simulink subsystem "cmac2d"  (R2024b)
settings: Solver=VariableStepAuto  StartTime=0.0  StopTime=10.0  RelTol=1e-3
undefined symbols (not defined in the file): Cin, Cout, L, LOG2L, NKEEP
libraries: hdlsllib x12
settings Model: Creator=User  LastModifiedBy=User

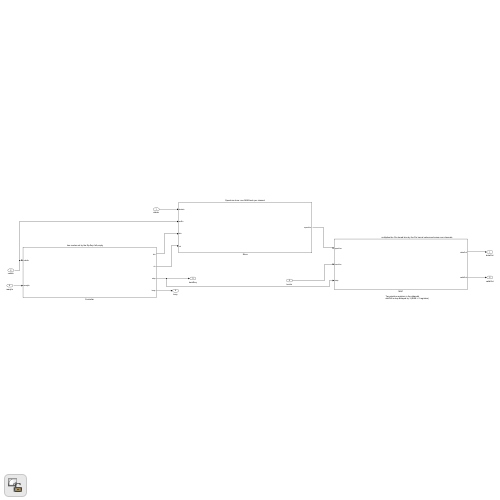
[thumbnail: Simulink's stored preview of the top-level diagram]
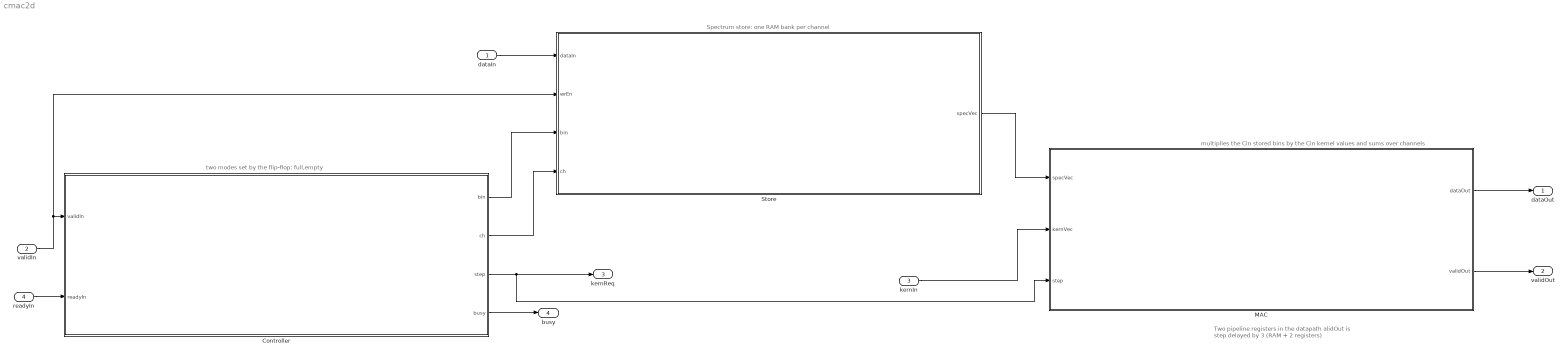
== system cmac2d ==
  note: two modes set by the flip-flop: full,empty
  note: Spectrum store: one RAM bank per channel
  note: multiplies the Cin stored bins by the Cin kernel values and sums over channels
  note: Two pipeline registers in the datapath
      | alidOut is step delayed by 3 (RAM + 2 registers)
  dataIn : Inport  OutDataTypeStr=fixdt(1,23,0)
      settings: SignalType=complex
  validIn : Inport  Port=2
  kernIn : Inport  Port=3  OutDataTypeStr=fixdt(1,KERN_WL,0)  PortDimensions=Cin
      settings: SignalType=complex
  readyIn : Inport  Port=4
  Controller : Subsystem
  MAC : Subsystem
  Store : Subsystem
  dataOut : Outport
  validOut : Outport  Port=2
  kernReq : Outport  Port=3
  busy : Outport  Port=4
  wires:
  Controller/3(step) -> kernReq/1, MAC/3(step)
  kernIn/1 -> MAC/2(kernVec)
  readyIn/1 -> Controller/2(readyIn)
  dataIn/1 -> Store/1(dataIn)
  validIn/1 -> Controller/1(validIn), Store/2(wrEn)
  Controller/1(bin) -> Store/3(bin)
  Controller/2(ch) -> Store/4(ch)
  Controller/4(busy) -> busy/1
  Store/1(specVec) -> MAC/1(specVec)
  MAC/1(dataOut) -> dataOut/1
  MAC/2(validOut) -> validOut/1

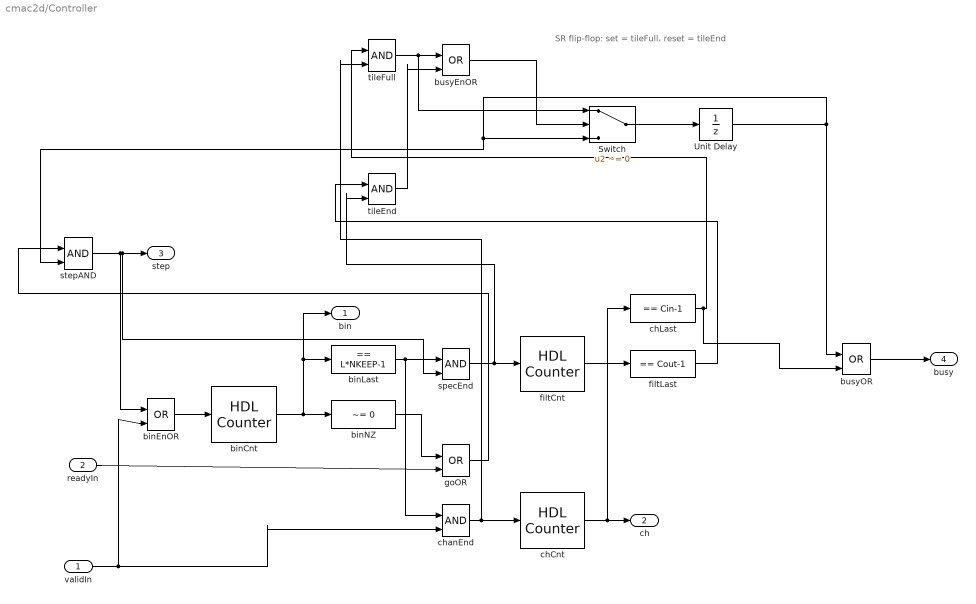
== system cmac2d/Controller ==
  note: SR flip-flop: set = tileFull، reset = tileEnd
  validIn : Inport
  readyIn : Inport  Port=2
  Switch : Switch  Criteria=u2 ~= 0  SaturateOnIntegerOverflow=off  InputSameDT=off
  Unit Delay : UnitDelay  SampleTime=-1  HasFrameUpgradeWarning=on
  binCnt : hdlsllib/Sources/HDL Counter  CountType=Count limited  CountInit=0  CountStep=1  CountMax=L*NKEEP-1  CountFromType=Initial value  CountFrom=0  CountResetPort=off  CountLoadPort=off  CountEnbPort=on  CountDirPort=off  CountHitOutputPort=off  CountDataType=Unsigned  CountWordLen=2*LOG2L  CountFracLen=0  CountSampTime=1
  binEnOR : Logic  Operator=OR  IconShape=distinctive  AllPortsSameDT=off  OutDataTypeStr=boolean
  binLast : hdlsllib/Logic and Bit Operations/Compare To Constant  relop===  const=L*NKEEP-1  OutDataTypeStr=boolean
  binNZ : hdlsllib/Logic and Bit Operations/Compare To Constant  relop=~=  const=0  OutDataTypeStr=boolean
  busyEnOR : Logic  Operator=OR  IconShape=distinctive  AllPortsSameDT=off  OutDataTypeStr=boolean
  busyOR : Logic  Operator=OR  IconShape=distinctive  AllPortsSameDT=off  OutDataTypeStr=boolean
  chCnt : hdlsllib/Sources/HDL Counter  CountType=Count limited  CountInit=0  CountStep=1  CountMax=Cin-1  CountFromType=Initial value  CountFrom=0  CountResetPort=off  CountLoadPort=off  CountEnbPort=on  CountDirPort=off  CountHitOutputPort=off  CountDataType=Unsigned  CountWordLen=ceil(log2(Cin))  CountFracLen=0  CountSampTime=1
  chLast : hdlsllib/Logic and Bit Operations/Compare To Constant  relop===  const=Cin-1  OutDataTypeStr=boolean
  chanEnd : Logic  IconShape=distinctive  AllPortsSameDT=off  OutDataTypeStr=boolean
  filtCnt : hdlsllib/Sources/HDL Counter  CountType=Count limited  CountInit=0  CountStep=1  CountMax=Cout-1  CountFromType=Initial value  CountFrom=0  CountResetPort=off  CountLoadPort=off  CountEnbPort=on  CountDirPort=off  CountHitOutputPort=off  CountDataType=Unsigned  CountWordLen=ceil(log2(Cout))  CountFracLen=0  CountSampTime=1
  filtLast : hdlsllib/Logic and Bit Operations/Compare To Constant  relop===  const=Cout-1  OutDataTypeStr=boolean
  goOR : Logic  Operator=OR  IconShape=distinctive  AllPortsSameDT=off  OutDataTypeStr=boolean
  specEnd : Logic  IconShape=distinctive  AllPortsSameDT=off  OutDataTypeStr=boolean
  stepAND : Logic  IconShape=distinctive  AllPortsSameDT=off  OutDataTypeStr=boolean
  tileEnd : Logic  IconShape=distinctive  AllPortsSameDT=off  OutDataTypeStr=boolean
  tileFull : Logic  IconShape=distinctive  AllPortsSameDT=off  OutDataTypeStr=boolean
  bin : Outport
  ch : Outport  Port=2
  step : Outport  Port=3
  busy : Outport  Port=4
  wires:
  busyOR/1 -> busy/1
  filtLast/1 -> tileEnd/1
  chLast/1 -> tileFull/1, busyOR/2
  chCnt/1 -> chLast/1, ch/1
  Switch/1 -> Unit Delay/1
  chanEnd/1 -> chCnt/1, tileFull/2
  busyEnOR/1 -> Switch/2
  goOR/1 -> stepAND/1
  readyIn/1 -> goOR/2
  binNZ/1 -> goOR/1
  tileEnd/1 -> busyEnOR/2
  tileFull/1 -> busyEnOR/1, Switch/1
  Unit Delay/1 -> stepAND/2, Switch/3, busyOR/1
  validIn/1 -> binEnOR/2, chanEnd/2
  specEnd/1 -> filtCnt/1, tileEnd/2
  binCnt/1 -> binNZ/1, bin/1, binLast/1
  binEnOR/1 -> binCnt/1
  binLast/1 -> chanEnd/1, specEnd/1
  stepAND/1 -> binEnOR/1, step/1, specEnd/2
  filtCnt/1 -> filtLast/1

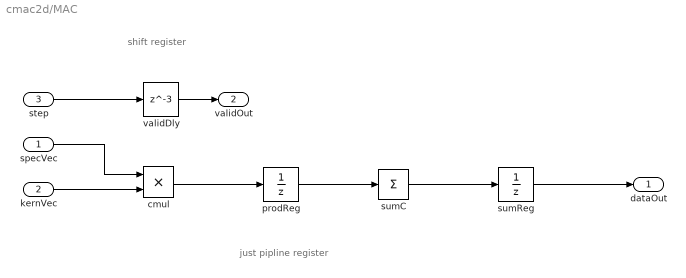
== system cmac2d/MAC ==
  note: just pipline register
  note: shift register
  specVec : Inport
  kernVec : Inport  Port=2
  step : Inport  Port=3
  cmul : Product  OutDataTypeStr=fixdt(1,X_WL+KERN_WL+1,0)
  prodReg : UnitDelay  SampleTime=-1  HasFrameUpgradeWarning=on
  sumC : Sum  Inputs=+  OutDataTypeStr=fixdt(1,X_WL+KERN_WL+1+ceil(log2(Cin)),0)
  sumReg : UnitDelay  SampleTime=-1  HasFrameUpgradeWarning=on
  validDly : Delay  DelayLength=3  InitialCondition=0
  dataOut : Outport
  validOut : Outport  Port=2
  wires:
  sumReg/1 -> dataOut/1
  prodReg/1 -> sumC/1
  validDly/1 -> validOut/1
  cmul/1 -> prodReg/1
  kernVec/1 -> cmul/2
  sumC/1 -> sumReg/1
  specVec/1 -> cmul/1
  step/1 -> validDly/1

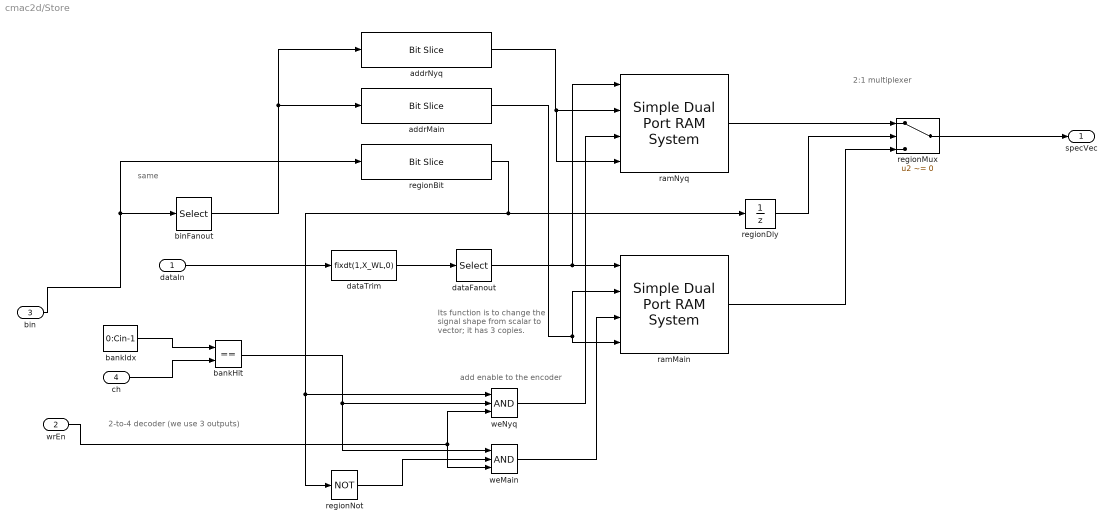
== system cmac2d/Store ==
  note: 2-to-4 decoder (we use 3 outputs)
  note: add enable to the encoder
  note: 2:1 multiplexer
  note: Its function is to change
      | the signal shape
      | from scalar to vector;
      |  it has 3 copies.
  note: same
  dataIn : Inport  PortDimensions=1
  wrEn : Inport  Port=2
  bin : Inport  Port=3
  ch : Inport  Port=4
  addrMain : hdlsllib/Logic and Bit Operations/Bit Slice  lidx=2*LOG2L-2  ridx=0
  addrNyq : hdlsllib/Logic and Bit Operations/Bit Slice  lidx=LOG2L-1  ridx=0
  bankHit : RelationalOperator  Operator===  OutDataTypeStr=boolean  InputSameDT=off
  bankIdx : Constant  Value=0:Cin-1  OutDataTypeStr=fixdt(0,ceil(log2(Cin)),0)
  binFanout : Selector  InputPortWidth=1  IndexOptions=Index vector (dialog)  Indices=ones(1,Cin)  OutputSizes=1
  dataFanout : Selector  InputPortWidth=1  IndexOptions=Index vector (dialog)  Indices=ones(1,Cin)  OutputSizes=1
  dataTrim : DataTypeConversion  OutDataTypeStr=fixdt(1,X_WL,0)  SaturateOnIntegerOverflow=off  RndMeth=Floor
  ramMain : hdlsllib/HDL RAMs/Simple Dual Port RAM System  RAMType=Simple dual port  AsyncRead=off  WriteOutputValue=New data  RAMInitialValue=0  allowBusInputs=off  WritesHaveOutput=on  NumReads=0  NumWrites=1  SimulateUsing=Code generation  ModelRAMDelay=on
  ramNyq : hdlsllib/HDL RAMs/Simple Dual Port RAM System  RAMType=Simple dual port  AsyncRead=off  WriteOutputValue=New data  RAMInitialValue=0  allowBusInputs=off  WritesHaveOutput=on  NumReads=0  NumWrites=1  SimulateUsing=Code generation  ModelRAMDelay=on
  regionBit : hdlsllib/Logic and Bit Operations/Bit Slice  lidx=2*LOG2L-1  ridx=2*LOG2L-1
  regionDly : UnitDelay  SampleTime=-1  HasFrameUpgradeWarning=on
  regionMux : Switch  Criteria=u2 ~= 0  SaturateOnIntegerOverflow=off  InputSameDT=off
  regionNot : Logic  Operator=NOT  IconShape=distinctive  AllPortsSameDT=off  OutDataTypeStr=boolean
  weMain : Logic  Inputs=3  IconShape=distinctive  AllPortsSameDT=off  OutDataTypeStr=boolean
  weNyq : Logic  Inputs=3  IconShape=distinctive  AllPortsSameDT=off  OutDataTypeStr=boolean
  specVec : Outport
  wires:
  regionDly/1 -> regionMux/2
  ramNyq/1 -> regionMux/1
  addrMain/1 -> ramMain/2, ramMain/4
  ramMain/1 -> regionMux/3
  dataFanout/1 -> ramNyq/1, ramMain/1
  weNyq/1 -> ramNyq/3
  addrNyq/1 -> ramNyq/4, ramNyq/2
  wrEn/1 -> weMain/3, weNyq/3
  weMain/1 -> ramMain/3
  bankHit/1 -> weNyq/2, weMain/1
  binFanout/1 -> addrNyq/1, addrMain/1
  regionMux/1 -> specVec/1
  ch/1 -> bankHit/2
  dataTrim/1 -> dataFanout/1
  regionBit/1 -> regionDly/1, weNyq/1, regionNot/1
  bankIdx/1 -> bankHit/1
  dataIn/1 -> dataTrim/1
  regionNot/1 -> weMain/2
  bin/1 -> binFanout/1, regionBit/1
